simulink model "hopper_6dof_NED_v2_fluid_integration"  (R2026a)
settings: Solver=FixedStepAuto  StopTime=tgrid(end)  FixedStep=1e-3  RelTol=1e-5
InitFcn:
  | load('FuelPropsData.mat');
undefined symbols (not defined in the file): cg_init, g, IN, K1flat, K2grid, OUT, r_leg_1, r_leg_2, r_leg_3, r_leg_4, Target_Trajectory, tgrid, unom, VEH
libraries: fl_lib x43, nesl_utility x31, SimscapeFluids_lib x13, matrix_library x9, slpidlib x3, simulink x3, simulink_extras x3, dspindex x1, aerolibanim x1, commrandsrc3 x1, aerolibutil x1, dspsrcs4 x1
(part 1 of 5)
settings Model: Creator=asing  LastModifiedBy=asing
settings DebuggingCC: SignalInfNanChecking=warning
settings SimscapeCC: SimscapeNominalValues="[{\"value\":\"1\",\"unit\":\"A\"},{\"value\":\"1\",\"unit\":\"bar\"},{\"value\":\"1\",\"unit\":\"cm^2\"},{\"value\":\"1\",\"unit\":\"cm^3/s\"},{\"value\":\"1\",\"unit\":\"kJ/kg\"},{\"value\":\"1\",\"unit\":\"kW\"},{\"value\":\"1\",\"unit\":\"l\"},{\"value\":\"1\",\"unit\":\"N\"},{\"value\":\"1\",\"unit\":\"N*m\"},{\"value\":\"1\",\"unit\":\"V\"}]"  SimscapeLogType=none  SimscapeLogDataHistory=5000.0

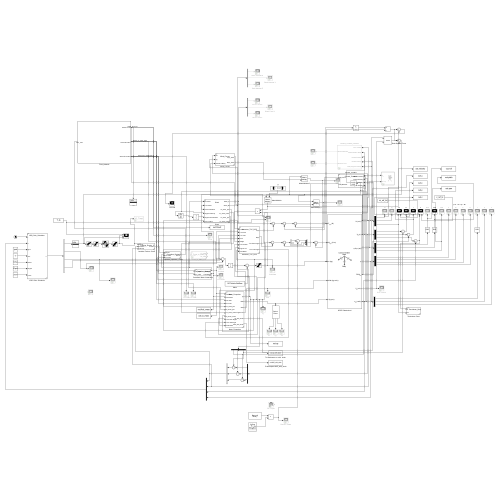
[thumbnail: Simulink's stored preview of the top-level diagram]
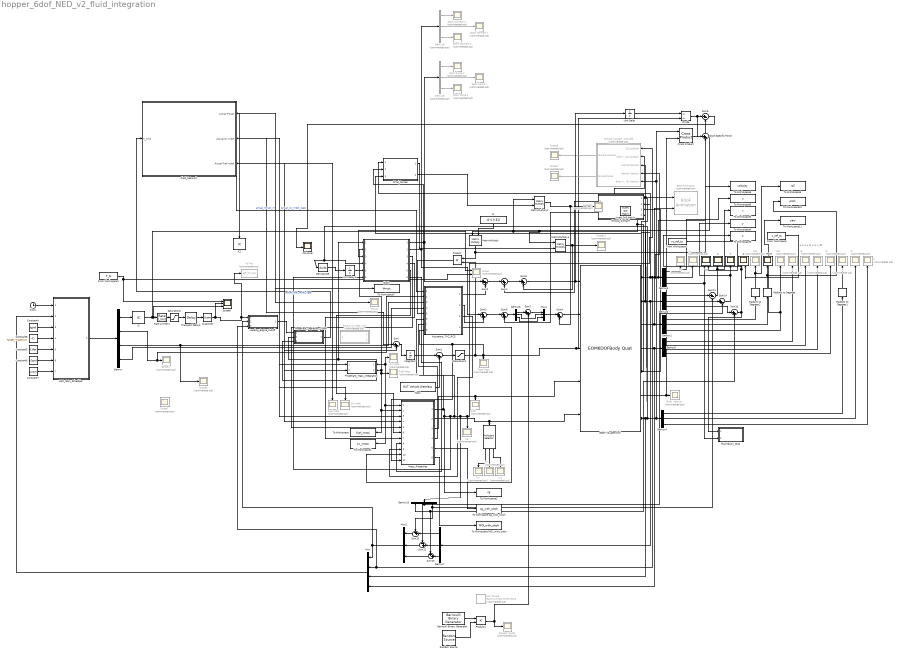
== system hopper_6dof_NED_v2_fluid_integration ==
  note: q = a + bi + cj + dk
  " " : dspindex/Multiport Selector  rowsOrCols=Rows  idxCellArray={1,2,3}  idxErrMode=Clip Index
      settings: LibrarySourceBlock=|
      | dsphdlsupportsigmgmt/Multiport
      | Selector
  6DOF (Quaternion) : EOM6DOFBodyQuat  mtype=Custom Variable  xme_0=[0 0 -cg_init]  eul_0=[0 pi/2 0]
  6DoF Animation : aerolibanim/6DoF Animation  Commented=on  u1=[0 200 -200 200 -100 5]  u2=0.1  u3=2  u4=[4000 0 -5000]  u5=Fly alongside  u6=[100 100 -50]  u7=10  u8=on
  A : Scope  Commented=on
      settings: ActiveDisplayYMinimum=-1  ActiveDisplayYMaximum=1  DataLoggingVariableName=ScopeData12
  Actuators_TVC_RCS : Subsystem  ReferencedSubsystem=Actuators_TVC_RCS
  B : Scope  Commented=on
      settings: ActiveDisplayYMinimum=-1  ActiveDisplayYMaximum=1  DataLoggingVariableName=ScopeData13
  Bernoulli Binary Generator : commrandsrc3/Bernoulli Binary Generator  ProbabilityOfZero=0.95  SeedSource=Parameter  Seed=0  SampleTime=0.1  SamplesPerFrame=1  OutputDataType=double  SimulateUsing=Interpreted execution
  Body Velocity : Scope  Commented=on
      settings: ActiveDisplayYMinimum=-9.910378836747423  ActiveDisplayYMaximum=88.214312640198585  DataLoggingVariableName=ScopeData29
  C : Scope  Commented=on
      settings: DataLoggingVariableName=ScopeData14
  CG Accel : Scope
      settings: ActiveDisplayYMinimum=-11.407629776225166  ActiveDisplayYMaximum=3.5948297727236085  DataLoggingVariableName=ScopeData33
  Clock : Clock
  Constant4 : Constant  Value=tgrid
  Constant5 : Constant  Value=K1flat
  Constant6 : Constant  Value=K2grid
  Constant7 : Constant  Value=unom
  Constant8 : Constant  Value=Target_Trajectory
  Cross Product : matrix_library/Cross Product
  D : Scope  Commented=on
      settings: DataLoggingVariableName=ScopeData15
  Demux : Demux
  Demux{1..4,6..7,10} (7 alike) : Demux  Outputs=3
  Demux5 : Demux
  Demux8 : Demux  Commented=on  Outputs=3
  Demux9 : Demux  Commented=on  Outputs=3
  Derivative3 : Derivative  CoefficientInTFapproximation=3
  Divide : Product  Inputs=*/
  Fluid_Network : Subsystem
  From Workspace : FromWorkspace  VariableName=z_ref_ts
  From Workspace1 : FromWorkspace  VariableName=T_ts
  From Workspace2 : FromWorkspace  VariableName=vz_ref_ts
  Fuel Mass : Scope  Commented=on
      settings: ActiveDisplayYMinimum=7.5154679010584076  ActiveDisplayYMaximum=13.609392455437956  DataLoggingVariableName=ScopeData18
  Fuel mdot : Scope  Commented=on
      settings: ActiveDisplayYMinimum=-0.057229294241176995  ActiveDisplayYMaximum=0.515142758459371  DataLoggingVariableName=ScopeData20
  Ground_Contact : Subsystem  ReferencedSubsystem=Ground_Contact
  Ground_Contact_Unwired : Subsystem  Commented=on
  IC : InitialCondition  Value=VEH.mass.wet*g
  IC1 : InitialCondition  Value=VEH.mass.wet*g
  Integrator : Integrator
  Invert 3x3 Matrix : aerolibutil/Invert  3x3 Matrix
  Ixx : Scope  Commented=on
      settings: ActiveDisplayYMinimum=-1.2693672305907171  ActiveDisplayYMaximum=1.7662706804264152  DataLoggingVariableName=ScopeData21
  Iyy : Scope  Commented=on
      settings: ActiveDisplayYMinimum=-8.2381488489345962  ActiveDisplayYMaximum=64.485305245521346  DataLoggingVariableName=ScopeData26
  Izz : Scope  Commented=on
      settings: ActiveDisplayYMinimum=-8.2393172969859414  ActiveDisplayYMaximum=64.3796161087634  DataLoggingVariableName=ScopeData27
  LQR_Gain_Scheduler : Subsystem  ReferencedSubsystem=LQR_Gain_Scheduler
  Landing_Engine_Cutoff : Subsystem  ReferencedSubsystem=Landing_Engine_Cutoff
  Mass : Constant  Value=OUT.Vehicle.WetMass
  Mass_Properties : Subsystem  ReferencedSubsystem=Mass_Properties
  MatrixMultiply : Product  Multiplication=Matrix(*)
  MatrixMultiply1 : Product  Multiplication=Matrix(*)
  MatrixMultiply2 : Product  Multiplication=Matrix(*)
  Mux : Mux
  Mux1 : Mux  Inputs=3
  Mux2 : Mux  Inputs=3
  Ox Mass : Scope  Commented=on
      settings: ActiveDisplayYMinimum=9.14433500982005  ActiveDisplayYMaximum=16.761740554464438  DataLoggingVariableName=ScopeData17
  Ox mdot : Scope  Commented=on
      settings: ActiveDisplayYMinimum=-0.071536617800839461  ActiveDisplayYMaximum=0.64392844807434468  DataLoggingVariableName=ScopeData19
  P : Scope  Commented=on
      settings: ActiveDisplayYMinimum=-40.272034282628653  ActiveDisplayYMaximum=40.18271139614702  DataLoggingVariableName=ScopeData9
  Pitch : Scope
      settings: ActiveDisplayYMinimum=43.438097555335354  ActiveDisplayYMaximum=90.504604934017451  DataLoggingVariableName=ScopeData4
  Product : Product
  Product1 : Product
  Propellant_Depletion_Cutoff : Subsystem  ReferencedSubsystem=Propellant_Depletion_Cutoff
  Propellant_Mass_Integration : Subsystem  ReferencedSubsystem=Propellant_Mass_Integration
  Q : Scope  Commented=on
      settings: ActiveDisplayYMinimum=-0.03908687484475059  ActiveDisplayYMaximum=0.052615482319584864  DataLoggingVariableName=ScopeData10
  Quantizer : Quantizer  QuantizationInterval=IN.throttle_valve.resolution
  R : Scope  Commented=on
      settings: ActiveDisplayYMinimum=-0.0070860969112896514  ActiveDisplayYMaximum=0.0085398632976064828  DataLoggingVariableName=ScopeData11
  Radians to Degrees : simulink_extras/Transformations/Radians to Degrees
  Radians to Degrees1 : simulink_extras/Transformations/Radians to Degrees
  Radians to Degrees2 : simulink_extras/Transformations/Radians to Degrees
  Random Source : dspsrcs4/Random Source  SrcType=Gaussian  MinVal=0  MaxVal=1  MeanVal=0  VarVal=20  RepMode=Specify seed  rawSeed=1  IsInherit=off  SampTime=1  SampFrame=1  OutComplex=Real  DataType=double  SimulateUsing=Interpreted execution
  Random Gusts : Scope  Commented=on
      settings: ActiveDisplayYMinimum=-8.5897961122323956  ActiveDisplayYMaximum=9.8055336087823335  DataLoggingVariableName=ScopeData63
  Rate Limiter1 : RateLimiter  RisingSlewLimit=IN.throttle_valve.rate_limit  FallingSlewLimit=-IN.throttle_valve.rate_limit  SampleTimeMode=inherited
  Roll : Scope  Commented=on
      settings: ActiveDisplayYMinimum=-204.65947396986587  ActiveDisplayYMaximum=175.17097918939032  DataLoggingVariableName=ScopeData3
  Roll Torque : simulink/Sources/Band-Limited White Noise  Commented=on  Cov=5  Ts=1  seed=[23341]
  Saturation1 : Saturate  UpperLimit=OUT.Vehicle.WetMass  LowerLimit=OUT.Vehicle.DryMass
  Saturation2 : Saturate  UpperLimit=IN.propulsion.nominal_thrust * IN.propulsion.throttle_range(2)  LowerLimit=IN.propulsion.nominal_thrust * IN.propulsion.throttle_range(1)
  Scope : Scope  Commented=on  NumInputPorts=2
      settings: ActiveDisplayYMinimum=725.64918679567745  ActiveDisplayYMaximum=1423.3753088923004  DataLoggingVariableName=ScopeData52
  Scope{1..3,5,7,11..12} (7 alike) : Scope  Commented=on
      Scope1 settings: ActiveDisplayYMinimum=-0.00050229611394169284  ActiveDisplayYMaximum=0.0028458999197228797  DataLoggingVariableName=ScopeData53
      Scope11 settings: ActiveDisplayYMinimum=-1.725572479086533  ActiveDisplayYMaximum=0.1917302754540588  DataLoggingVariableName=ScopeData66
      Scope12 settings: ActiveDisplayYMinimum=-2.88543679656206  ActiveDisplayYMaximum=6.7910588943113428  DataLoggingVariableName=ScopeData67
      Scope2 settings: ActiveDisplayYMinimum=-8449.52436564975  ActiveDisplayYMaximum=76045.719290847759  DataLoggingVariableName=ScopeData49
      Scope3 settings: ActiveDisplayYMinimum=-903.54597657114152  ActiveDisplayYMaximum=89.720851920197276  DataLoggingVariableName=ScopeData51
      Scope5 settings: ActiveDisplayYMinimum=-0.0014807269526439936  ActiveDisplayYMaximum=0.00063209871075060983  DataLoggingVariableName=ScopeData57
      Scope7 settings: ActiveDisplayYMinimum=-9.3466701964128269  ActiveDisplayYMaximum=8.508922841651323  DataLoggingVariableName=ScopeData62
  Scope6 : Scope  NumInputPorts=3
      settings: ActiveDisplayYMinimum=-12632.794590273525  ActiveDisplayYMaximum=4410.2403285914115  DataLoggingVariableName=ScopeData59
  Slosh : Subsystem  ReferencedSubsystem=Slosh
  Slosh Force X : Scope  Commented=on
      settings: ActiveDisplayYMinimum=-23.703787957912279  ActiveDisplayYMaximum=30.843704332518367  DataLoggingVariableName=ScopeData32
  Slosh Force Y : Scope  Commented=on
      settings: ActiveDisplayYMinimum=-0.5552642189596475  ActiveDisplayYMaximum=0.52836332227705041  DataLoggingVariableName=ScopeData72
  Slosh Force Z : Scope  Commented=on
      settings: ActiveDisplayYMinimum=-0.4568274165323904  ActiveDisplayYMaximum=0.43197139726332079  DataLoggingVariableName=ScopeData73
  Slosh Moment X : Scope  Commented=on
      settings: ActiveDisplayYMinimum=-1  ActiveDisplayYMaximum=1  DataLoggingVariableName=ScopeData74
  Slosh Moment Y : Scope  Commented=on
      settings: ActiveDisplayYMinimum=-0.020821390947241118  ActiveDisplayYMaximum=0.019580844558623325  DataLoggingVariableName=ScopeData75
  Slosh Moment Z : Scope  Commented=on
      settings: ActiveDisplayYMinimum=-0.045380586631965543  ActiveDisplayYMaximum=0.048640802204673789  DataLoggingVariableName=ScopeData76
  Slosh Specific Force : Sum  Description=(F_total/m) - g_body = non-gravitational specific force at the CG; drives the slosh pendulums.  Inputs=|+-
  Sum{,2..5,7..9,15} (9 alike) : Sum  Inputs=|++
  Sum1 : Sum  Inputs=|-+
  Sum10 : Sum  Inputs=-+|
  Sum11 : Sum  Inputs=|+-
  Sum12 : Sum  Inputs=-+|
  Sum13 : Sum  Inputs=++|
  Sum14 : Sum  Inputs=|+-
  Sum6 : Sum  Inputs=|+-
  Thrust : Scope  Commented=on
      settings: ActiveDisplayYMinimum=-212.49999999999994  ActiveDisplayYMaximum=1912.5  DataLoggingVariableName=ScopeData25
  Thrust_to_Mdot_LUT : Subsystem  Commented=on  ReferencedSubsystem=Thrust_to_Mdot_LUT
  To File : ToFile  Commented=on  Filename=AP_T.mat  SaveFormat=Timeseries
  To Workspace : ToWorkspace  VariableName=fuel_mass  SaveFormat=Timeseries  SampleTime=-1
  To Workspace MOI_with_slosh : ToWorkspace  VariableName=MOI_with_slosh  SaveFormat=Timeseries  SampleTime=-1
  To Workspace cg_with_slosh : ToWorkspace  VariableName=cg_with_slosh  SaveFormat=Timeseries  SampleTime=-1
  To Workspace1 : ToWorkspace  VariableName=ox_mass  SaveFormat=Timeseries  SampleTime=-1
  To Workspace10 : ToWorkspace  VariableName=pitch  SaveFormat=Timeseries  SampleTime=-1
  To Workspace11 : ToWorkspace  VariableName=yaw  SaveFormat=Timeseries  SampleTime=-1
  To Workspace2 : ToWorkspace  VariableName=cg  SaveFormat=Timeseries  SampleTime=-1
  To Workspace3 : ToWorkspace  VariableName=x  SaveFormat=Timeseries  SampleTime=-1
  To Workspace4 : ToWorkspace  VariableName=y  SaveFormat=Timeseries  SampleTime=-1
  To Workspace5 : ToWorkspace  VariableName=z  SaveFormat=Timeseries  SampleTime=-1
  To Workspace6 : ToWorkspace  VariableName=u  SaveFormat=Timeseries  SampleTime=-1
  To Workspace7 : ToWorkspace  VariableName=thrust  SaveFormat=Timeseries  SampleTime=-1
  To Workspace8 : ToWorkspace  VariableName=velocity  SaveFormat=Timeseries  SampleTime=-1
  To Workspace9 : ToWorkspace  VariableName=roll  SaveFormat=Timeseries  SampleTime=-1
  Total Mass : Scope  Commented=on
      settings: ActiveDisplayYMinimum=123.40007682459402  ActiveDisplayYMaximum=148.35554701948959  DataLoggingVariableName=ScopeData16
  Touchdown_Stop : Subsystem  ReferencedSubsystem=Touchdown_Stop
  Transport Delay2 : TransportDelay  DelayTime=IN.throttle_valve_latency
  Unit Delay : UnitDelay  SampleTime=-1
  Unit Delay1 : UnitDelay  SampleTime=-1
  Vx : Scope  Commented=on
      settings: ActiveDisplayYMinimum=-1.0568314607793221  ActiveDisplayYMaximum=0.63247821872235255  DataLoggingVariableName=ScopeData6
  Vy : Scope  Commented=on
      settings: ActiveDisplayYMinimum=-1  ActiveDisplayYMaximum=1  DataLoggingVariableName=ScopeData7
  Vz : Scope  NumInputPorts=2
      settings: ActiveDisplayYMinimum=-0.40844386646617703  ActiveDisplayYMaximum=1.313724578805866  DataLoggingVariableName=ScopeData8
  Wind_Forces : Subsystem  ReferencedSubsystem=Wind_Forces
  X : Scope
      settings: ActiveDisplayYMinimum=-0.57285266608571106  ActiveDisplayYMaximum=0.60376762362057124
  Y : Scope
      settings: ActiveDisplayYMinimum=-0.45246190447103363  ActiveDisplayYMaximum=0.388758387694069
  Yaw : Scope  Commented=on
      settings: ActiveDisplayYMinimum=-0.29772085399940185  ActiveDisplayYMaximum=2.6794861130407197  DataLoggingVariableName=ScopeData5
  Z : Scope  NumInputPorts=2
      settings: ActiveDisplayYMinimum=-0.11627941832016962  ActiveDisplayYMaximum=0.086760786687265876  DataLoggingVariableName=ScopeData2
  cg : Scope  Commented=on
      settings: ActiveDisplayYMinimum=-0.21955738430461946  ActiveDisplayYMaximum=1.426543136357856  DataLoggingVariableName=ScopeData23
  dI/dt : Scope  Commented=on
      settings: ActiveDisplayYMinimum=-0.25764178573017943  ActiveDisplayYMaximum=0.028626865081131041  DataLoggingVariableName=ScopeData22
  g : Constant  Value=[0 0 9.81]
  wires:
  6DOF (Quaternion)/2 -> Ground_Contact_Unwired/3(Inertial Position), 6DoF Animation/1, Demux2/1, Demux7/1, Ground_Contact/1
  6DOF (Quaternion)/3 -> 6DoF Animation/2, Demux1/1
  Demux1/2 -> Radians to Degrees/1
  Demux3/1 -> To Workspace6/1, Vx/1
  Demux3/2 -> Vy/1
  6DOF (Quaternion)/4 -> Mux/4, Demux5/1
  Demux4/1 -> Radians to Degrees1/1
  Demux4/2 -> Q/1
  Demux4/3 -> R/1
  Demux5/1 -> A/1
  Demux5/2 -> B/1
  Demux5/3 -> C/1
  Demux5/4 -> D/1
  Demux3/3 -> Touchdown_Stop/2, Vz/1
  Sum/1 -> Integrator/1
  Integrator/1 -> Sum1/1
  Mass/1 -> Sum1/2
  Sum1/1 -> Saturation1/1
  Saturation1/1 -> Actuators_TVC_RCS/8, Mass_Properties/11, Divide/2, 6DOF (Quaternion)/3, Total Mass/1, Product/2
  Propellant_Mass_Integration/2 -> Propellant_Depletion_Cutoff/3, Slosh/2, Fuel Mass/1, To Workspace/1, Mass_Properties/2
  Mass_Properties/2 -> 6DOF (Quaternion)/5, " "/1
  Mass_Properties/3 -> 6DOF (Quaternion)/4, dI/dt/1
  Actuators_TVC_RCS/1 -> Sum2/2
  Actuators_TVC_RCS/2 -> Sum3/2
  Propellant_Mass_Integration/1 -> Propellant_Depletion_Cutoff/2, Slosh/1, To Workspace1/1, Mass_Properties/1, Ox Mass/1
  6DOF (Quaternion)/6 -> Cross Product/2, Body Velocity/1
  MatrixMultiply/1 -> Product/1, Slosh Specific Force/2
  Invert 3x3 Matrix/1 -> Ground_Contact_Unwired/2(DCM Inertial to Body)
  Sum2/1 -> Sum4/1
  Sum3/1 -> Sum5/1
  Cross Product/1 -> Sum6/2
  Divide/1 -> Sum6/1, Slosh Specific Force/1
  Sum6/1 -> CG Accel/1
  Unit Delay/1 -> Divide/1
  Ground_Contact_Unwired/2(Ground Force) -> Scope2/1
  Ground_Contact_Unwired/1(Ground Moment) -> Scope3/1
  Slosh/2 -> Sum3/1, Demux9/1
  Slosh/1 -> Demux8/1, Sum2/1
  Derivative3/1 -> Unit Delay1/1
  Product/1 -> Actuators_TVC_RCS/5
  Demux1/1 -> Radians to Degrees2/1
  Demux1/3 -> Yaw/1, To Workspace11/1
  g/1 -> MatrixMultiply/2
  Rate Limiter1/1 -> Saturation2/1
  Demux/2 -> Actuators_TVC_RCS/2, Scope1/1
  Demux/3 -> Actuators_TVC_RCS/3, Scope5/1
  Demux/1 -> IC/1
  Transport Delay2/1 -> Quantizer/1
  From Workspace1/1 -> Scope6/1, Scope/2
  IC/1 -> Scope/1, Scope6/3, Rate Limiter1/1
  From Workspace2/1 -> Vz/2
  Sum7/1 -> Mux1/1
  Demux6/1 -> Sum7/1
  Demux6/2 -> Mux1/2
  Demux6/3 -> Mux1/3
  Sum5/1 -> Demux6/1
  Wind_Forces/2 -> MatrixMultiply2/2
  6DOF (Quaternion)/1 -> Wind_Forces/1, Landing_Engine_Cutoff/3, Mux/2, Ground_Contact_Unwired/4(Inertial Velocity), To Workspace8/1, Demux3/1, Ground_Contact/2
  Sum8/1 -> Unit Delay/1, 6DOF (Quaternion)/1
  Sum4/1 -> Sum8/1
  Mux1/1 -> Sum9/1
  Sum9/1 -> 6DOF (Quaternion)/2
  6DOF (Quaternion)/5 -> MatrixMultiply1/1, MatrixMultiply2/1, MatrixMultiply/1, Invert 3x3 Matrix/1, Wind_Forces/3, Ground_Contact/3
  Wind_Forces/1 -> MatrixMultiply1/2
  MatrixMultiply1/1 -> Sum8/2, Scope11/1
  MatrixMultiply2/1 -> Sum9/2, Scope12/1
  Mux2/1 -> Mux/1, Landing_Engine_Cutoff/2
  Mass_Properties/1 -> Wind_Forces/2, To Workspace2/1, Slosh/6, Demux10/1, Ground_Contact_Unwired/1(CG Location), cg/1, Actuators_TVC_RCS/6
  Demux8/1 -> Slosh Force X/1
  Demux8/2 -> Slosh Force Y/1
  Demux8/3 -> Slosh Force Z/1
  Demux9/1 -> Slosh Moment X/1
  Demux9/2 -> Slosh Moment Y/1
  Demux9/3 -> Slosh Moment Z/1
  Landing_Engine_Cutoff/1 -> Propellant_Depletion_Cutoff/1
  Saturation2/1 -> Transport Delay2/1
  Quantizer/1 -> Scope6/2, Landing_Engine_Cutoff/1, To File/1
  6DOF (Quaternion)/7 -> Mux/3, Ground_Contact_Unwired/5(Body Angular Velocity), Cross Product/1, Demux4/1, Derivative3/1, Slosh/4, Ground_Contact/4
  Demux7/1 -> Sum10/2
  Sum10/1 -> Mux2/1
  Sum12/1 -> Mux2/2
  Demux7/2 -> Sum12/2
  Demux7/3 -> Sum13/2
  Sum13/1 -> Mux2/3
  Demux10/2 -> Sum14/2, Sum12/1
  Demux10/3 -> Sum11/2, Sum10/1
  Demux10/1 -> Sum15/2, Sum13/1
  Demux2/1 -> Sum11/1
  Sum11/1 -> To Workspace3/1, X/1
  Demux2/2 -> Sum14/1
  Sum14/1 -> To Workspace4/1, Y/1
  Demux2/3 -> Sum15/1
  Slosh/3 -> Mass_Properties/5
  Slosh/4 -> Mass_Properties/7
  Slosh/5 -> Mass_Properties/6
  Slosh/6 -> Mass_Properties/8
  Actuators_TVC_RCS/3 -> Mass_Properties/9
  Actuators_TVC_RCS/4 -> Mass_Properties/10
  Mass_Properties/4 -> Actuators_TVC_RCS/7
  " "/1 -> Ixx/1
  " "/2 -> Iyy/1
  " "/3 -> Izz/1
  Unit Delay1/1 -> Slosh/5
  Demux/4 -> Actuators_TVC_RCS/4
  Radians to Degrees/1 -> To Workspace10/1, Pitch/1
  Sum15/1 -> To Workspace5/1, Z/1, Touchdown_Stop/1
  From Workspace/1 -> Z/2
  Bernoulli Binary Generator/1 -> Product1/1
  Random Source/1 -> Product1/2
  Product1/1 -> Sum7/2, Random Gusts/1
  Radians to Degrees1/1 -> P/1
  Radians to Degrees2/1 -> To Workspace9/1, Roll/1
  Slosh Specific Force/1 -> Slosh/3
  Mass_Properties/5 -> To Workspace cg_with_slosh/1
  Mass_Properties/6 -> To Workspace MOI_with_slosh/1
  Clock/1 -> LQR_Gain_Scheduler/1
  Mux/1 -> LQR_Gain_Scheduler/2
  Constant4/1 -> LQR_Gain_Scheduler/3
  Constant8/1 -> LQR_Gain_Scheduler/4
  Constant5/1 -> LQR_Gain_Scheduler/5
  Constant6/1 -> LQR_Gain_Scheduler/6
  Constant7/1 -> LQR_Gain_Scheduler/7
  LQR_Gain_Scheduler/1 -> Demux/1
  Propellant_Depletion_Cutoff/1 -> Fluid_Network/1(F_cmd)
  Fluid_Network/1(Actual Thrust) -> IC1/1, Actuators_TVC_RCS/1, To Workspace7/1, Thrust/1  "actual_thrust_N"
  Fluid_Network/2(Actual Ox mdot) -> Sum/1, Propellant_Mass_Integration/1, Mass_Properties/3, Ox mdot/1  "actual_ox_mdot_kgps"
  Fluid_Network/3(Actual Fuel mdot) -> Sum/2, Propellant_Mass_Integration/2, Fuel mdot/1, Mass_Properties/4  "actual_fuel_mdot_kgps"
  Ground_Contact/1 -> Sum4/2
  Ground_Contact/2 -> Sum5/2

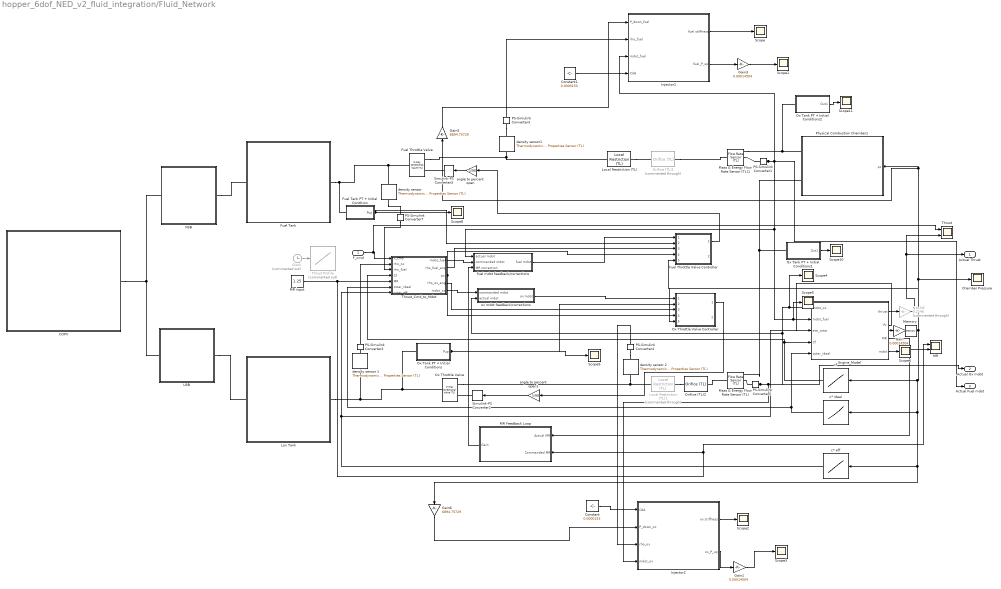
== system hopper_6dof_NED_v2_fluid_integration/Fluid_Network ==
  F_cmd : Inport
  COPV : Subsystem
  Chamber Pressure : Scope
      settings: ActiveDisplayYMinimum=24.4768520913143  ActiveDisplayYMaximum=276.14956071215624  DataLoggingVariableName=ScopeData22
  Clock : Clock  Commented=on
  Constant : Constant  Value=0.0000153
  Constant1 : Constant  Value=0.0000153
  Engine_Model : MATLAB Function  TreatAsAtomicUnit=on
  FBB : Subsystem
  Fuel Tank : Subsystem
  Fuel Tank PT + Initial Condition : Subsystem
  Fuel Throttle Valve : SimscapeFluids_lib/Thermal Liquid/Valves & Orifices/Directional Control Valves/2-Way Directional Valve (TL)  valve_spec=fluids.thermal_liquid.valves.directional_control_valves.enum.ValveSpec.Table1DAreaOpening  S_max=1 m  del_S_max=5e-3 m  area_max=1e-4 m^2  area_leak=1e-10 m^2  del_S_TLU=[0 0.3 0.4 0.5 0.6 0.7 0.8 0.9 1.0] m  valve_area_TLU=[1e-9 1.7065e-07 1.0239e-06 3.5836e-06 7.8498e-06 1.4164e-05 2.3038e-05 3.4812e-05 5.0000e-05] m^2  del_S_flow_TLU=[0, .002, .004, .007, .017] m  p_diff_TLU=[.3, .5, .7] MPa  vol_flow_TLU=1e-3 * [1.7e-05, 2e-05, 2.6e-05; .0035, .0045, .0053; .7, .9, 1.06; 1.96, 2.5, 3; 6, 7.7, 9.13] m^3/s  mdot_TLU=[1.7e-05, 2e-05, 2.6e-05; .0035, .0045, .0053; .7, .9, 1.06; 1.96, 2.5, 3; 6, 7.7, 9.13] kg/s  T_ref_in=293.15 K  p_ref_in=0.101325 MPa  Cd=1  Re_c=150  smoothing_factor=0.01  pressure_recovery=false  area=0.01 m^2
  Fuel Throttle Valve Controller : Subsystem  ReferencedSubsystem=Throttle_Valve_Controller  ramp_slope=60
  Gain : Gain  Gain=0.00014504
  Gain1 : Gain  Gain=0.00014504
  Gain3 : Gain  Gain=0.00014504
  Gain5 : Gain  Gain=6894.75729
  Gain6 : Gain  Gain=6894.75729
  Injector1 : Subsystem
  Injector2 : Subsystem
  LBB : Subsystem
  Local Restriction (TL) : fl_lib/Thermal Liquid/Elements/Local Restriction (TL)  restriction_type=foundation.enum.restriction_type.fixed  restriction_area=0.0000153 m^2  min_area=1e-10 m^2  max_area=0.005 m^2  area=0.000153 m^2  Cd=1  Re_c=150  pressure_recovery=true
  Local Restriction (TL)1 : fl_lib/Thermal Liquid/Elements/Local Restriction (TL)  Commented=through  restriction_type=foundation.enum.restriction_type.fixed  restriction_area=0.0000153 m^2  min_area=1e-10 m^2  max_area=0.005 m^2  area=0.000153 m^2  Cd=1  Re_c=150  pressure_recovery=true
  Lox Tank : Subsystem
  MR : Scope  NumInputPorts=2
      settings: ActiveDisplayYMinimum=0.081947452963374467  ActiveDisplayYMaximum=2.5817499803566988
  MR Feedback Loop : Subsystem
  MR input : Constant  Value=1.25
  Mass & Energy Flow Rate Sensor (TL) : fl_lib/Thermal Liquid/Sensors/Flow Rate Sensor (TL)  mass_flow_measure=true  volumetric_flow_measure=false  energy_flow_measure=true
  Mass & Energy Flow Rate Sensor (TL)1 : fl_lib/Thermal Liquid/Sensors/Flow Rate Sensor (TL)  mass_flow_measure=true  volumetric_flow_measure=false  energy_flow_measure=true
  Memory : Memory  InitialCondition=300
  N to lbf : Gain  Commented=through  Gain=0.2248
  Orifice (TL)1 : SimscapeFluids_lib/Thermal Liquid/Valves & Orifices/Orifice (TL)  Commented=through  orifice_type=foundation.enum.constant_variable.constant  constant_orifice_spec=fluids.thermal_liquid.valves.enum.ConstantOrificeSpec.Area  variable_orifice_spec=fluids.thermal_liquid.valves.enum.orifice_spec.linear  orifice_area_constant=0.0000153 m^2  p_diff_TLU_constant=[-4, -3, -2, -1, -.5, 0, .5, 1, 2, 3, 4] MPa  vol_flow_TLU_constant=[-2.44, -2.12, -1.68, -1.22, -.84, 0, .85, 1.21, 1.7, 2.09, 2.41] .* 1e-3 m^3/s  mdot_TLU_constant=[-2.44, -2.12, -1.68, -1.22, -.84, 0, .85, 1.21, 1.7, 2.09, 2.41] kg/s  S_min=0 m  del_S=5e-3 m  open_orientation=fluids.thermal_liquid.valves.enum.orifice_orientation.positive  area_max=1e-4 m^2  area_leak=1e-10 m^2  S_TLU=[0, .002, .004, .007, .017] m  orifice_area_TLU=[1e-09, 2.0352e-07, 4.0736e-05, .00011438, .00034356] m^2  Cd=1  Re_c=150  smoothing_factor=0.01  pressure_recovery=false  S_flow_TLU=[0, .002, .004, .007, .017] m  p_diff_TLU=[.3, .5, .7] MPa  vol_flow_TLU=1e-3 * [1.7e-05, 2e-05, 2.6e-05; .0035, .0045, .0053; .7, .9, 1.06; 1.96, 2.5, 3; 6, 7.7, 9.13] m^3/s  mdot_TLU=[1.7e-05, 2e-05, 2.6e-05; .0035, .0045, .0053; .7, .9, 1.06; 1.96, 2.5, 3; 6, 7.7, 9.13] kg/s  T_ref_in=293.15 K  p_ref_in=0.101325 MPa  area=0.01 m^2
  Orifice (TL)2 : SimscapeFluids_lib/Thermal Liquid/Valves & Orifices/Orifice (TL)  orifice_type=foundation.enum.constant_variable.constant  constant_orifice_spec=fluids.thermal_liquid.valves.enum.ConstantOrificeSpec.Area  variable_orifice_spec=fluids.thermal_liquid.valves.enum.orifice_spec.linear  orifice_area_constant=0.0000153 m^2  p_diff_TLU_constant=[-4, -3, -2, -1, -.5, 0, .5, 1, 2, 3, 4] MPa  vol_flow_TLU_constant=[-2.44, -2.12, -1.68, -1.22, -.84, 0, .85, 1.21, 1.7, 2.09, 2.41] .* 1e-3 m^3/s  mdot_TLU_constant=[-2.44, -2.12, -1.68, -1.22, -.84, 0, .85, 1.21, 1.7, 2.09, 2.41] kg/s  S_min=0 m  del_S=5e-3 m  open_orientation=fluids.thermal_liquid.valves.enum.orifice_orientation.positive  area_max=1e-4 m^2  area_leak=1e-10 m^2  S_TLU=[0, .002, .004, .007, .017] m  orifice_area_TLU=[1e-09, 2.0352e-07, 4.0736e-05, .00011438, .00034356] m^2  Cd=1  Re_c=150  smoothing_factor=0.01  pressure_recovery=false  S_flow_TLU=[0, .002, .004, .007, .017] m  p_diff_TLU=[.3, .5, .7] MPa  vol_flow_TLU=1e-3 * [1.7e-05, 2e-05, 2.6e-05; .0035, .0045, .0053; .7, .9, 1.06; 1.96, 2.5, 3; 6, 7.7, 9.13] m^3/s  mdot_TLU=[1.7e-05, 2e-05, 2.6e-05; .0035, .0045, .0053; .7, .9, 1.06; 1.96, 2.5, 3; 6, 7.7, 9.13] kg/s  T_ref_in=293.15 K  p_ref_in=0.101325 MPa  area=0.01 m^2
  Ox Tank PT + Initial Conditions : Subsystem
  Ox Tank PT + Initial Conditions1 : Subsystem
  Ox Tank PT + Initial Conditions2 : Subsystem
  Ox Throttle Valve : SimscapeFluids_lib/Thermal Liquid/Valves & Orifices/Directional Control Valves/2-Way Directional Valve (TL)  valve_spec=fluids.thermal_liquid.valves.directional_control_valves.enum.ValveSpec.Table1DAreaOpening  S_max=1 m  del_S_max=5e-3 m  area_max=1e-4 m^2  area_leak=1e-10 m^2  del_S_TLU=[0 0.3 0.4 0.5 0.6 0.7 0.8 0.9 1.0] m  valve_area_TLU=[1e-9 1.7065e-07 1.0239e-06 3.5836e-06 7.8498e-06 1.4164e-05 2.3038e-05 3.4812e-05 5.0000e-05] m^2  del_S_flow_TLU=[0, .002, .004, .007, .017] m  p_diff_TLU=[.3, .5, .7] MPa  vol_flow_TLU=1e-3 * [1.7e-05, 2e-05, 2.6e-05; .0035, .0045, .0053; .7, .9, 1.06; 1.96, 2.5, 3; 6, 7.7, 9.13] m^3/s  mdot_TLU=[1.7e-05, 2e-05, 2.6e-05; .0035, .0045, .0053; .7, .9, 1.06; 1.96, 2.5, 3; 6, 7.7, 9.13] kg/s  T_ref_in=293.15 K  p_ref_in=0.101325 MPa  Cd=1  Re_c=150  smoothing_factor=0.01  pressure_recovery=false  area=0.01 m^2
  Ox Throttle Valve Controller : Subsystem  ReferencedSubsystem=Throttle_Valve_Controller  ramp_slope=48
  PS-Simulink Converter{1..5,7} (6 alike) : nesl_utility/PS-Simulink Converter  PhysicalDomain=network_engine_domain  SubClassName=ps_output  LeftPortType=input  RightPortType=output  PseudoPeriodic=off  Frequencies=[]  VectorFormat=inherit  Unit=inherit  AffineConversion=off
  Physical Combustion Chamber1 : Subsystem
  Scope{,1..6,8..11} (11 alike) : Scope
      Scope settings: ActiveDisplayYMinimum=-0.024254245068718681  ActiveDisplayYMaximum=0.21828827495285463  DataLoggingVariableName=ScopeData40
      Scope1 settings: ActiveDisplayYMinimum=-37.465424615708343  ActiveDisplayYMaximum=337.50135970832162  DataLoggingVariableName=ScopeData42
      Scope10 settings: ActiveDisplayYMinimum=-62.731329785992315  ActiveDisplayYMaximum=586.85713455527571  DataLoggingVariableName=ScopeData51
      Scope11 settings: ActiveDisplayYMinimum=-62.499971643181283  ActiveDisplayYMaximum=562.49999684924239  DataLoggingVariableName=ScopeData52
      Scope2 settings: ActiveDisplayYMinimum=-0.025857157768165939  ActiveDisplayYMaximum=0.4462125176132366  DataLoggingVariableName=ScopeData43
      Scope3 settings: ActiveDisplayYMinimum=-1  ActiveDisplayYMaximum=1  DataLoggingVariableName=ScopeData44
      Scope4 settings: ActiveDisplayYMinimum=-0.071595374751251564  ActiveDisplayYMaximum=0.64519605918641931  DataLoggingVariableName=ScopeData53
      Scope5 settings: ActiveDisplayYMinimum=-0.05515719954820638  ActiveDisplayYMaximum=0.49713967255882957  DataLoggingVariableName=ScopeData54
      Scope6 settings: ActiveDisplayYMinimum=-0.1205205125313115  ActiveDisplayYMaximum=1.086247175831931  DataLoggingVariableName=ScopeData55
      Scope8 settings: ActiveDisplayYMinimum=481.05362935967628  ActiveDisplayYMaximum=536.06057249536832  DataLoggingVariableName=ScopeData49
      Scope9 settings: ActiveDisplayYMinimum=492.10107740407369  ActiveDisplayYMaximum=524.51908611925091  DataLoggingVariableName=ScopeData50
  Simulink-PS Converter2 : nesl_utility/Simulink-PS Converter  PhysicalDomain=network_engine_domain  SubClassName=ps_input  LeftPortType=input  RightPortType=output  PseudoPeriodic=off  Frequencies=[]  NoiseDistribution=none  NoiseParameters=[]  Unit=1  AffineConversion=off  FilteringAndDerivatives=filter  SimscapeFilterOrder=1  InputFilterTimeConstant=0.001  UdotUserProvided=0
  Simulink-PS Converter3 : nesl_utility/Simulink-PS Converter  PhysicalDomain=network_engine_domain  SubClassName=ps_input  LeftPortType=input  RightPortType=output  PseudoPeriodic=off  Frequencies=[]  NoiseDistribution=none  NoiseParameters=[]  Unit=1  AffineConversion=off  FilteringAndDerivatives=filter  SimscapeFilterOrder=1  InputFilterTimeConstant=0.001  UdotUserProvided=0
  Thrust : Scope  NumInputPorts=2
      settings: ActiveDisplayYMinimum=-215.53569406218494  ActiveDisplayYMaximum=1942.1553478833205  DataLoggingVariableName=ScopeData21
  Thrust Profile : Lookup_n-D  Commented=on  NumberOfTableDimensions=1  BreakpointsForDimension1=|  Table=|  InternalRulePriority=Speed  RndMeth=Simplest
      BreakpointsForDimension1=|
      | [0
      | 2.46e-15
      | 4.93e-15
      | 1.31e-14
      | 1.85798e-4
      | 3.71595e-4
      | 1.300583e-3
      | 5.945524e-3
      | 2.917023e-2
      | 1.452937e-1
      | 3.251823e-1
      | 6.176896e-1
      | 1.048884
      | 1.648122
      | 2.452841
      | 3.452841
      | 4.452841
      | 5.452841
      | 6.452841
      | 7.452841
      | 8.452841
      | 9.452841
      | 10.45284
      | 11.45284
      | 12.45284
      | 13.45284
      | 14.45284
      | 15.45284
      | 16.26888
      | 17.26888
      | 18.26888
      | 19.26888
      | 20.26888
      | 21.26888
      | 21.82014
      | 22.37140
      | 23.10183
      | 24.10183
      | 25.10183
      | 26.10183
      | 27.10183
      | 28.10183
      | 29.10183
      | 29.70287]
      Table=|
      | [1115.929794
      | 1115.929794
      | 1115.929794
      | 1115.929794
      | 1116.015031
      | 1116.100248
      | 1116.526042
      | 1118.647732
      | 1129.075722
      | 1176.888468
      | 1237.984070
      | 1309.087819
      | 1365.657208
      | 1382.500173
      | 1347.869214
      | 1276.732855
      | 1209.886660
      | 1007.359221
      | 890.000000
      | 890.000000
      | 890.000000
      | 890.000000
      | 970.372958
      | 1015.368113
      | 1034.720854
      | 1040.888013
      | 1040.596927
      | 896.870767
      | 890.000000
      | 890.000000
      | 890.000000
      | 890.000000
      | 890.000000
      | 890.000000
      | 1074.062231
      | 1213.486737
      | 1218.338865
      | 1172.384789
      | 1114.978943
      | 1066.195681
      | 1030.043331
      | 1004.841448
      | 987.599936
      | 979.912878]
  Thrust_Cmd_to_Mdot : MATLAB Function  TreatAsAtomicUnit=on
  angle to percent open : Gain  Gain=1/90
  angle to percent open1 : Gain  Gain=1/90
  c* eff : Lookup_n-D  NumberOfTableDimensions=1  BreakpointsForDimension1=[125 295]  Table=[0.8 0.85]  InternalRulePriority=Speed  RndMeth=Simplest
  c* ideal : Lookup_n-D  NumberOfTableDimensions=1  BreakpointsForDimension1=[100 110 120 130 140 150 160 170 180 190 200 210 220 230 240 250 260 270 280 290 300 310 320 330 340 350]  Table=[1492.810749 1492.812678 1492.815823 1492.820080 1492.825344 1492.831574 1492.838703 1492.846662 1492.855462 1492.865052 1492.875406 1492.886504 1492.898325 1492.910854 1492.924078 1492.937982 1492.952558 1492.967791 1492.983688 1493.000184 1493.017345 1493.035113 1493.053494 1493.072480 1493.092063 1493.112237]  InternalRulePriority=Speed  RndMeth=Simplest
  cf : Lookup_n-D  NumberOfTableDimensions=1  BreakpointsForDimension1=[125 295]  Table=[1.42 1.57]  InternalRulePriority=Speed  RndMeth=Simplest
  density sensor : fl_lib/Thermal Liquid/Sensors/Thermodynamic Properties Sensor (TL)  internal_energy=false  density=true  specific_heat=false
  density sensor 1 : fl_lib/Thermal Liquid/Sensors/Thermodynamic Properties Sensor (TL)  internal_energy=false  density=true  specific_heat=false
  density sensor 2 : fl_lib/Thermal Liquid/Sensors/Thermodynamic Properties Sensor (TL)  internal_energy=false  density=true  specific_heat=false
  density sensor1 : fl_lib/Thermal Liquid/Sensors/Thermodynamic Properties Sensor (TL)  internal_energy=false  density=true  specific_heat=false
  fuel mdot feedback/corrections : Subsystem
  ox mdot feedback/corrections : Subsystem
  Actual Thrust : Outport
  Actual Ox mdot : Outport  Port=2
  Actual Fuel mdot : Outport  Port=3
  wires:
  c* ideal/1 -> Engine_Model/5(cstar_ideal), Thrust_Cmd_to_Mdot/6(cstar_ideal)
  Fuel Tank PT + Initial Condition/1(Pup) -> Scope8/1, Fuel Throttle Valve Controller/2
  N to lbf/1 -> Thrust/2, Actual Thrust/1
  Thrust_Cmd_to_Mdot/1(mdot_fuel) -> fuel mdot feedback/corrections/2(commanded mdot)
  Ox Tank PT + Initial Conditions/1(Pup) -> Scope9/1, Ox Throttle Valve Controller/2
  angle to percent open/1 -> Simulink-PS Converter3/1
  angle to percent open1/1 -> Simulink-PS Converter2/1
  Engine_Model/3(MR) -> MR Feedback Loop/1(Actual MR), MR/2
  Thrust_Cmd_to_Mdot/5(mdot_ox) -> ox mdot feedback/corrections/1(commanded mdot)
  Clock/1 -> Thrust Profile/1
  Engine_Model/1(thrust) -> N to lbf/1
  Gain/1 -> Memory/1
  Engine_Model/2(Pc) -> Gain/1
  MR Feedback Loop/1(Gain) -> fuel mdot feedback/corrections/3(MR correction)
  MR input/1 -> MR Feedback Loop/2(Commanded MR), MR/1, Thrust_Cmd_to_Mdot/5(MR)
  Thrust_Cmd_to_Mdot/3(pc) -> Fuel Throttle Valve Controller/4, Ox Throttle Valve Controller/4
  PS-Simulink Converter2/1 -> Thrust_Cmd_to_Mdot/2(rho_ox)
  c* eff/1 -> Thrust_Cmd_to_Mdot/7(cstar_eff), Engine_Model/3(eta_cstar)
  cf/1 -> Thrust_Cmd_to_Mdot/4(Cf), Engine_Model/4(Cf)
  F_cmd/1 -> Thrust/1, Thrust_Cmd_to_Mdot/1(F_cmd)
  PS-Simulink Converter5/1 -> Actual Ox mdot/1, Injector2/4(mdot_ox), Scope4/1, Engine_Model/1(mdot_ox), ox mdot feedback/corrections/2(actual mdot)
  PS-Simulink Converter1/1 -> Actual Fuel mdot/1, Injector1/3(mdot_fuel), Scope5/1, Engine_Model/2(mdot_fuel), fuel mdot feedback/corrections/1(actual mdot)
  Injector1/1(fuel stiffness) -> Scope/1
  Injector1/2(fuel_P_up) -> Gain3/1
  Injector2/1(ox stiffness) -> Scope2/1
  Injector2/2(ox_P_up) -> Gain1/1
  Constant/1 -> Injector2/1(CdA)
  Constant1/1 -> Injector1/4(CdA)
  PS-Simulink Converter7/1 -> Thrust_Cmd_to_Mdot/3(rho_fuel)
  Ox Tank PT + Initial Conditions1/1(Out1) -> Scope10/1
  Ox Tank PT + Initial Conditions2/1(Out1) -> Scope11/1
  Gain3/1 -> Scope1/1
  Gain1/1 -> Scope3/1
  Gain5/1 -> Injector1/1(P_down_fuel)
  Gain6/1 -> Injector2/2(P_down_ox)
  Memory/1 -> Gain6/1, c* eff/1, c* ideal/1, cf/1, Gain5/1, Physical Combustion Chamber1/1(pc), Chamber Pressure/1, Fuel Throttle Valve Controller/5, Ox Throttle Valve Controller/5
  PS-Simulink Converter3/1 -> Injector1/2(rho_fuel)
  PS-Simulink Converter4/1 -> Injector2/3(rho_ox)
  Engine_Model/4(mdot) -> Scope6/1
  fuel mdot feedback/corrections/1(fuel mdot) -> Fuel Throttle Valve Controller/1
  Thrust_Cmd_to_Mdot/2(rho_fuel_eng) -> Fuel Throttle Valve Controller/3
  Fuel Throttle Valve Controller/1 -> angle to percent open/1
  ox mdot feedback/corrections/1(ox mdot) -> Ox Throttle Valve Controller/1
  Thrust_Cmd_to_Mdot/4(rho_ox_eng) -> Ox Throttle Valve Controller/3
  Ox Throttle Valve Controller/1 -> angle to percent open1/1
  connections:
  density sensor 1/RConn1 -- PS-Simulink Converter2/LConn1
  LBB/RConn1 -- Lox Tank/LConn1
  Fuel Tank/RConn1 -- Fuel Throttle Valve/LConn1 -- density sensor/LConn1 -- Fuel Tank PT + Initial Condition/LConn1
  Simulink-PS Converter3/RConn1 -- Fuel Throttle Valve/RConn1
  PS-Simulink Converter5/LConn1 -- Mass & Energy Flow Rate Sensor (TL)/RConn2
  Ox Throttle Valve/RConn2 -- Local Restriction (TL)1/LConn1 -- density sensor 2/LConn1
  Mass & Energy Flow Rate Sensor (TL)1/RConn1 -- Physical Combustion Chamber1/RConn1 -- Ox Tank PT + Initial Conditions2/LConn1
  FBB/RConn1 -- Fuel Tank/LConn1
  Ox Tank PT + Initial Conditions1/LConn1 -- Physical Combustion Chamber1/RConn2 -- Mass & Energy Flow Rate Sensor (TL)/RConn1
  density sensor/RConn1 -- PS-Simulink Converter7/LConn1
  Lox Tank/RConn1 -- density sensor 1/LConn1 -- Ox Tank PT + Initial Conditions/LConn1 -- Ox Throttle Valve/LConn1
  COPV/RConn1 -- LBB/LConn1 -- FBB/LConn1
  PS-Simulink Converter1/LConn1 -- Mass & Energy Flow Rate Sensor (TL)1/RConn2
  Simulink-PS Converter2/RConn1 -- Ox Throttle Valve/RConn1
  Fuel Throttle Valve/RConn2 -- density sensor1/LConn1 -- Local Restriction (TL)/LConn1
  Orifice (TL)1/RConn1 -- Mass & Energy Flow Rate Sensor (TL)1/LConn1
  Orifice (TL)2/RConn1 -- Mass & Energy Flow Rate Sensor (TL)/LConn1
  PS-Simulink Converter3/LConn1 -- density sensor1/RConn1
  PS-Simulink Converter4/LConn1 -- density sensor 2/RConn1
  Local Restriction (TL)/RConn1 -- Orifice (TL)1/LConn1
  Local Restriction (TL)1/RConn1 -- Orifice (TL)2/LConn1

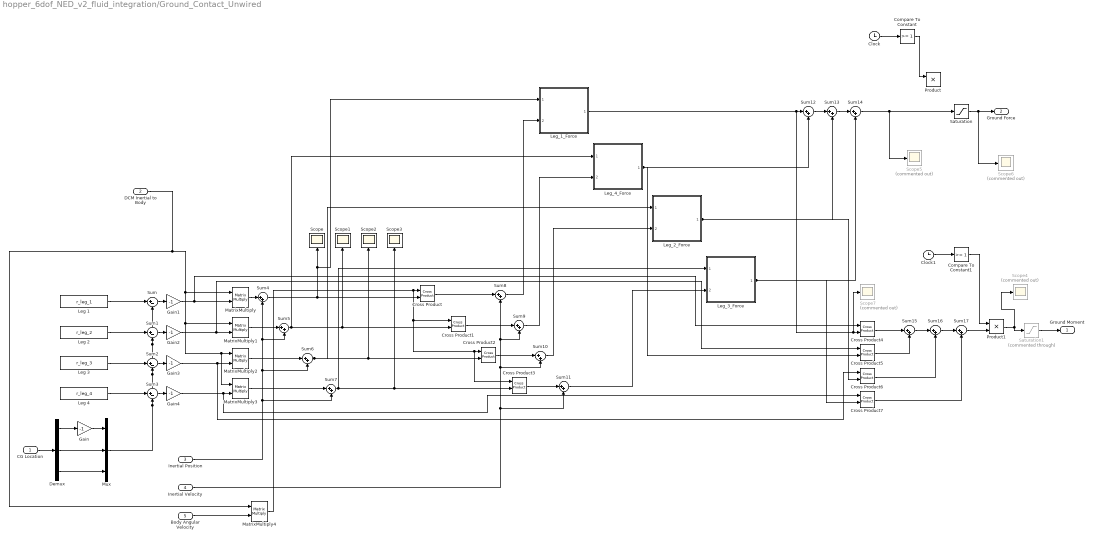
== system hopper_6dof_NED_v2_fluid_integration/Ground_Contact_Unwired ==
  CG Location : Inport
  DCM Inertial to Body : Inport  Port=2
  Inertial Position : Inport  Port=3
  Inertial Velocity : Inport  Port=4
  Body Angular Velocity : Inport  Port=5
  Clock : Clock
  Clock1 : Clock
  Compare To Constant : simulink/Logic and Bit Operations/Compare To Constant  relop=>=  const=1  OutDataTypeStr=boolean
  Compare To Constant1 : simulink/Logic and Bit Operations/Compare To Constant  relop=>=  const=1  OutDataTypeStr=boolean
  Cross Product{,1..7} (8 alike) : matrix_library/Cross Product
  Demux : Demux  Outputs=3
  Gain{,1..4} (5 alike) : Gain  Gain=-1
  Leg 1 : Constant  Value=r_leg_1
  Leg 2 : Constant  Value=r_leg_2
  Leg 3 : Constant  Value=r_leg_3
  Leg 4 : Constant  Value=r_leg_4
  Leg_1_Force : Subsystem  ReferencedSubsystem=Leg_Force_Unwired
  Leg_2_Force : Subsystem  ReferencedSubsystem=Leg_Force_Unwired
  Leg_3_Force : Subsystem  ReferencedSubsystem=Leg_Force_Unwired
  Leg_4_Force : Subsystem  ReferencedSubsystem=Leg_Force_Unwired
  MatrixMultiply{,1..4} (5 alike) : Product  Multiplication=Matrix(*)
  Mux : Mux  Inputs=3
  Product : Product
  Product1 : Product
  Saturation : Saturate  UpperLimit=inf  LowerLimit=0
  Saturation1 : Saturate  Commented=through  UpperLimit=inf  LowerLimit=0
  Scope{,1..3} (4 alike) : Scope
      Scope settings: ActiveDisplayYMinimum=-19.811154048207108  ActiveDisplayYMaximum=167.31101950999761  DataLoggingVariableName=ScopeData24
      Scope1 settings: ActiveDisplayYMinimum=182.10765195211306  ActiveDisplayYMaximum=183.93696889205802  DataLoggingVariableName=ScopeData30
      Scope2 settings: DataLoggingVariableName=ScopeData31
      Scope3 settings: DataLoggingVariableName=ScopeData42
  Scope{4..7} (4 alike) : Scope  Commented=on
      Scope4 settings: ActiveDisplayYMinimum=-3.0293963365637429E+7  ActiveDisplayYMaximum=2.2731893212350109E+8  DataLoggingVariableName=ScopeData43
      Scope5 settings: ActiveDisplayYMinimum=-31343.151613259419  ActiveDisplayYMaximum=282088.36451933486  DataLoggingVariableName=ScopeData44
      Scope6 settings: ActiveDisplayYMinimum=-136.62925150266653  ActiveDisplayYMaximum=1229.6632635239991  DataLoggingVariableName=ScopeData45
      Scope7 settings: ActiveDisplayYMinimum=-3.5823523450793636E+8  ActiveDisplayYMaximum=5.8466661508525646E+8  DataLoggingVariableName=ScopeData61
  Sum{,1..3} (4 alike) : Sum  Inputs=|+-
  Sum{4..17} (14 alike) : Sum  Inputs=|++
  Ground Moment : Outport
  Ground Force : Outport  Port=2
  wires:
  Demux/2 -> Mux/2
  Demux/3 -> Mux/3
  Leg 1/1 -> Sum/1
  Leg 2/1 -> Sum1/1
  Leg 3/1 -> Sum2/1
  Leg 4/1 -> Sum3/1
  Mux/1 -> Sum3/2, Sum1/2, Sum/2, Sum2/2
  Sum/1 -> Gain1/1
  DCM Inertial to Body/1 -> MatrixMultiply4/1, MatrixMultiply1/1, MatrixMultiply3/1, MatrixMultiply2/1, MatrixMultiply/1
  Sum1/1 -> Gain2/1
  Sum2/1 -> Gain3/1
  Sum3/1 -> Gain4/1
  MatrixMultiply3/1 -> Sum7/1
  MatrixMultiply2/1 -> Sum6/1
  MatrixMultiply1/1 -> Sum5/1
  MatrixMultiply/1 -> Sum4/1
  Inertial Position/1 -> Sum7/2, Sum6/2, Sum5/2, Sum4/2
  Sum4/1 -> Scope/1, Leg_1_Force/1, Cross Product/2
  Sum5/1 -> Scope1/1, Cross Product1/2, Leg_4_Force/1
  Sum6/1 -> Scope2/1, Cross Product2/2, Leg_2_Force/1
  Sum7/1 -> Scope3/1, Cross Product3/2, Leg_3_Force/1
  Body Angular Velocity/1 -> MatrixMultiply4/2
  MatrixMultiply4/1 -> Cross Product1/1, Cross Product3/1, Cross Product2/1, Cross Product/1
  Cross Product/1 -> Sum8/1
  Cross Product1/1 -> Sum9/1
  Cross Product2/1 -> Sum10/1
  Cross Product3/1 -> Sum11/1
  Inertial Velocity/1 -> Sum11/2, Sum10/2, Sum9/2, Sum8/2
  Leg_1_Force/1 -> Scope7/1, Cross Product4/2, Sum12/1
  Sum12/1 -> Sum13/1
  Sum13/1 -> Sum14/1
  Cross Product4/1 -> Sum15/1
  Sum15/1 -> Sum16/1
  Cross Product5/1 -> Sum15/2
  Cross Product6/1 -> Sum16/2
  Sum16/1 -> Sum17/1
  Cross Product7/1 -> Sum17/2
  Sum8/1 -> Leg_1_Force/2
  Saturation/1 -> Ground Force/1, Scope6/1
  Saturation1/1 -> Ground Moment/1
  Gain/1 -> Mux/1
  Gain1/1 -> Cross Product4/1, MatrixMultiply/2
  Gain2/1 -> Cross Product5/1, MatrixMultiply1/2
  Gain3/1 -> Cross Product6/1, MatrixMultiply2/2
  Gain4/1 -> Cross Product7/1, MatrixMultiply3/2
  Sum14/1 -> Saturation/1, Scope5/1
  Clock1/1 -> Compare To Constant1/1
  Compare To Constant1/1 -> Product1/1
  Sum17/1 -> Product1/2
  Product1/1 -> Scope4/1, Saturation1/1
  CG Location/1 -> Demux/1
  Demux/1 -> Gain/1
  Clock/1 -> Compare To Constant/1
  Compare To Constant/1 -> Product/1
  Sum10/1 -> Leg_2_Force/2
  Leg_2_Force/1 -> Cross Product6/2, Sum13/2
  Sum11/1 -> Leg_3_Force/2
  Leg_3_Force/1 -> Cross Product7/2, Sum14/2
  Sum9/1 -> Leg_4_Force/2
  Leg_4_Force/1 -> Cross Product5/2, Sum12/2
